simulink model "3. To develop elementary signals Unit step signal, unit ramp signal, unit impulse signal, exponential signal."  (R2024b)
settings: Solver=VariableStepAuto  StartTime=0.0  StopTime=10.0  RelTol=1e-3  EnableMultiTasking=on
libraries: dspsrcs4 x1, simulink x1
settings Model: Creator=CSE  LastModifiedBy=sobha
settings SolverCC: AlgebraicLoopSolver=TrustRegion
settings DataIOCC: ReturnWorkspaceOutputs=off
settings OptimizationCC: LifeSpan=inf
settings DebuggingCC: UnconnectedInputMsg=warning  UnconnectedOutputMsg=warning  UnconnectedLineMsg=warning  SFUnexpectedBacktrackingDiag=warning  SFNoUnconditionalDefaultTransitionDiag=warning  ArithmeticOperatorsInVariantConditions=warning
settings ModelReferenceCC: EnableRefExpFcnMdlSchedulingChecks=on
settings SFSimCC: SimUseLocalCustomCode=off  CustomCodeUndefinedFunction=UseInterfaceOnly
settings RTWCC: RTWUseLocalCustomCode=off  GPUComputeCapability=3.5
settings CodeAppCC: StateflowObjectComments=on
settings GRTTargetCC: TargetLangStandard=C89/C90 (ANSI)
settings ConfigComp: CovMetricSettings=dw  CovSaveCumulativeToWorkspaceVar=on  CovSaveSingleToWorkspaceVar=on  CovExternalEMLEnable=off

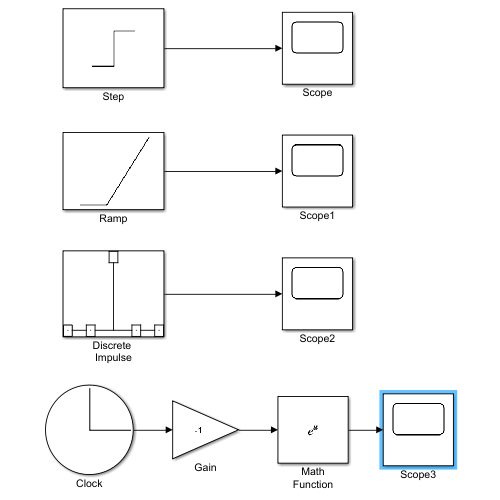
[thumbnail: Simulink's stored preview of the top-level diagram]
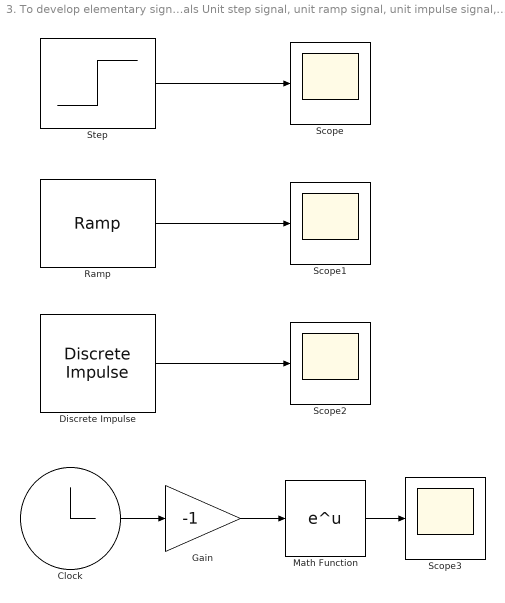
== system 3. To develop elementary signals Unit step signal, unit ramp signal, unit impulse signal, exponential signal. ==
  Clock : Clock
  Discrete Impulse : dspsrcs4/Discrete  Impulse  Delay=3  SampleTime=1  FrameSample=1  OutputFrames=off  dataType=double  isSigned=on  wordLen=16  udDataType=sfix(16)  fracBitsMode=Best precision  numFracBits=15  OutDataTypeStr=double  LastOutDataTypeStr=double
  Gain : Gain  Gain=-1
  Math Function : Math  SignedPower=on
  Ramp : simulink/Sources/Ramp  slope=1  start=0  InitialOutput=0
  Scope{,1..3} (4 alike) : Scope
  Step : Step  SampleTime=0
  wires:
  Step/1 -> Scope/1
  Ramp/1 -> Scope1/1
  Discrete Impulse/1 -> Scope2/1
  Clock/1 -> Gain/1
  Gain/1 -> Math Function/1
  Math Function/1 -> Scope3/1
